simulink model "nonlinearfinal"  (R2021b)
settings: Solver=VariableStepAuto  StartTime=0.0  StopTime=10.0  RelTol=1e-3
libraries: slpidlib x2
settings Model: Creator=Arian  LastModifiedBy=Arian

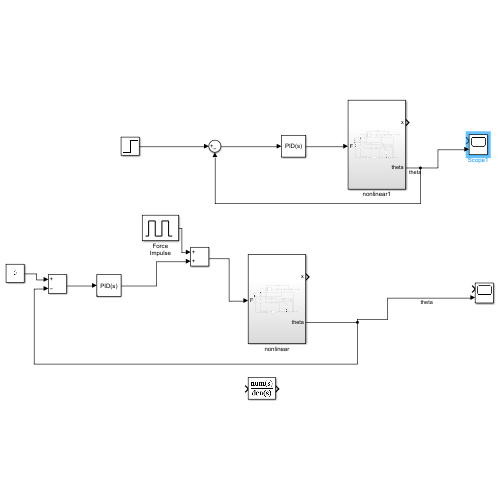
[thumbnail: Simulink's stored preview of the top-level diagram]
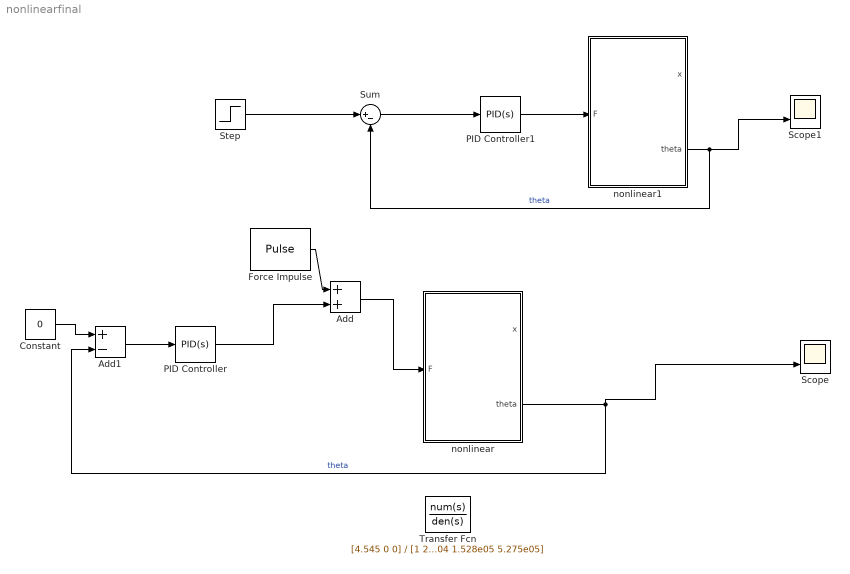
== system nonlinearfinal ==
  Add : Sum
  Add1 : Sum  Inputs=+-
  Constant : Constant  Value=0
  Force Impulse : DiscretePulseGenerator  PulseType=Time based  Amplitude=1000  Period=10  PulseWidth=0.01
  PID Controller : slpidlib/PID Controller  Controller=PID  Form=Parallel  TimeDomain=Continuous-time  UseExternalTs=off  SampleTime=-1  IntegratorMethod=Forward Euler  FilterMethod=Forward Euler  ControllerParametersSource=internal  P=100  I=100  D=20  UseFilter=on  N=1000  TunerSelectOption=Transfer Function Based (PID Tuner App)  InitialConditionSource=internal  InitialConditionForIntegrator=0  InitialConditionForFilter=0  DifferentiatorICPrevScaledInput=0  ExternalReset=none  TrackingMode=off  Kt=1  LimitOutput=off  SatLimitsSource=internal  UpperSaturationLimit=inf  LowerSaturationLimit=-inf  LinearizeAsGain=on  AntiWindupMode=none  Kb=1  POutMin=[]  POutMax=[]  IOutMin=[]  IOutMax=[]  DOutMin=[]  DOutMax=[]  NOutMin=[]  NOutMax=[]  SumOutMin=[]  SumOutMax=[]  SaturationOutMin=[]  SaturationOutMax=[]  PParamMin=[]  PParamMax=[]  IParamMin=[]  IParamMax=[]  DParamMin=[]  DParamMax=[]  NParamMin=[]  NParamMax=[]  KbParamMin=[]  KbParamMax=[]  KtParamMin=[]  KtParamMax=[]  KbOutMin=[]  KbOutMax=[]  KtOutMin=[]  KtOutMax=[]  IntegratorOutMin=[]  IntegratorOutMax=[]  FilterOutMin=[]  FilterOutMax=[]  SumI1OutMin=[]  SumI1OutMax=[]  SumI2OutMin=[]  SumI2OutMax=[]  SumI3OutMin=[]  SumI3OutMax=[]  SumI4OutMin=[]  SumI4OutMax=[]  SumDOutMin=[]  SumDOutMax=[]  DifferentiatorOutMin=[]  DifferentiatorOutMax=[]  FilterDiffOutCoefMin=[]  FilterDiffOutCoefMax=[]  ReciprocalOutMin=[]  ReciprocalOutMax=[]  SumDenOutMin=[]  SumDenOutMax=[]  SumNumOutMin=[]  SumNumOutMax=[]  DivideOutMin=[]  DivideOutMax=[]  UdiffTsProdOutMin=[]  UdiffTsProdOutMax=[]  NTsProdOutMin=[]  NTsProdOutMax=[]  UintegralTsProdOutMin=[]  UintegralTsProdOutMax=[]  UngainTsProdOutMin=[]  UngainTsProdOutMax=[]  IntegratorContinuousStateAttributes=''  IntegratorStateMustResolveToSignalObject=off  IntegratorRTWStateStorageClass=Auto  FilterContinuousStateAttributes=''  FilterStateMustResolveToSignalObject=off  FilterRTWStateStorageClass=Auto  ParallelPVariant=InternalParameters  IdealPVariant=Disabled  IVariant=InternalParameters  DVariant=InternalParameters  IntegratorVariant=Continuous  SatVariant=Disabled  AWVariant=Passthrough  PCopyVariant=Disabled  TRVariant=Disabled  FdbkBlocksVariant=Forward  IdealPFdbkVariant=Disabled  SatFdbkVariant=Disabled  DerivativeFilterVariant=ContFilter  NVariant=InternalParameters  NCopyVariant=Disabled  FilterICVariant=InternalICsFilter  IntegratorICVariant=InternalICs  ExternalResetVariant=Disabled  TRSumVariant=Passthrough  SumFdbkVariant=Disabled  SumVariant=Sum_PID  TsampFilterVariant=InternalTs  TsampNgainVariant=Passthrough  TsampIntegralVariant=Passthrough  ExternalSaturationOutDataTypeStr=Inherit: Same as second input
  PID Controller1 : slpidlib/PID Controller  Controller=PID  Form=Parallel  TimeDomain=Continuous-time  UseExternalTs=off  SampleTime=-1  IntegratorMethod=Forward Euler  FilterMethod=Forward Euler  ControllerParametersSource=internal  P=100  I=100  D=20  UseFilter=on  N=100  TunerSelectOption=Transfer Function Based (PID Tuner App)  InitialConditionSource=internal  InitialConditionForIntegrator=0  InitialConditionForFilter=0  DifferentiatorICPrevScaledInput=0  ExternalReset=none  TrackingMode=off  Kt=1  LimitOutput=off  SatLimitsSource=internal  UpperSaturationLimit=inf  LowerSaturationLimit=-inf  LinearizeAsGain=on  AntiWindupMode=none  Kb=1  POutMin=[]  POutMax=[]  IOutMin=[]  IOutMax=[]  DOutMin=[]  DOutMax=[]  NOutMin=[]  NOutMax=[]  SumOutMin=[]  SumOutMax=[]  SaturationOutMin=[]  SaturationOutMax=[]  PParamMin=[]  PParamMax=[]  IParamMin=[]  IParamMax=[]  DParamMin=[]  DParamMax=[]  NParamMin=[]  NParamMax=[]  KbParamMin=[]  KbParamMax=[]  KtParamMin=[]  KtParamMax=[]  KbOutMin=[]  KbOutMax=[]  KtOutMin=[]  KtOutMax=[]  IntegratorOutMin=[]  IntegratorOutMax=[]  FilterOutMin=[]  FilterOutMax=[]  SumI1OutMin=[]  SumI1OutMax=[]  SumI2OutMin=[]  SumI2OutMax=[]  SumI3OutMin=[]  SumI3OutMax=[]  SumI4OutMin=[]  SumI4OutMax=[]  SumDOutMin=[]  SumDOutMax=[]  DifferentiatorOutMin=[]  DifferentiatorOutMax=[]  FilterDiffOutCoefMin=[]  FilterDiffOutCoefMax=[]  ReciprocalOutMin=[]  ReciprocalOutMax=[]  SumDenOutMin=[]  SumDenOutMax=[]  SumNumOutMin=[]  SumNumOutMax=[]  DivideOutMin=[]  DivideOutMax=[]  UdiffTsProdOutMin=[]  UdiffTsProdOutMax=[]  NTsProdOutMin=[]  NTsProdOutMax=[]  UintegralTsProdOutMin=[]  UintegralTsProdOutMax=[]  UngainTsProdOutMin=[]  UngainTsProdOutMax=[]  IntegratorContinuousStateAttributes=''  IntegratorStateMustResolveToSignalObject=off  IntegratorRTWStateStorageClass=Auto  FilterContinuousStateAttributes=''  FilterStateMustResolveToSignalObject=off  FilterRTWStateStorageClass=Auto  ParallelPVariant=InternalParameters  IdealPVariant=Disabled  IVariant=InternalParameters  DVariant=InternalParameters  IntegratorVariant=Continuous  SatVariant=Disabled  AWVariant=Passthrough  PCopyVariant=Disabled  TRVariant=Disabled  FdbkBlocksVariant=Forward  IdealPFdbkVariant=Disabled  SatFdbkVariant=Disabled  DerivativeFilterVariant=ContFilter  NVariant=InternalParameters  NCopyVariant=Disabled  FilterICVariant=InternalICsFilter  IntegratorICVariant=InternalICs  ExternalResetVariant=Disabled  TRSumVariant=Passthrough  SumFdbkVariant=Disabled  SumVariant=Sum_PID  TsampFilterVariant=InternalTs  TsampNgainVariant=Passthrough  TsampIntegralVariant=Passthrough  ExternalSaturationOutDataTypeStr=Inherit: Same as second input
  Scope : Scope  NumInputPorts=2
  Scope1 : Scope  NumInputPorts=2
  Step : Step  SampleTime=0
  Sum : Sum  Inputs=|+-
  Transfer Fcn : TransferFcn  Numerator=[4.545 0 0]  Denominator=[1 250 1.68e04 1.528e05 5.275e05]
  nonlinear : Subsystem
  nonlinear1 : Subsystem
  wires:
  nonlinear1/2(theta) -> Scope1/2, Sum/2  "theta"
  PID Controller1/1 -> nonlinear1/1(F)
  Sum/1 -> PID Controller1/1
  Step/1 -> Sum/1
  Add1/1 -> PID Controller/1
  Constant/1 -> Add1/1
  Add/1 -> nonlinear/1(F)
  PID Controller/1 -> Add/2
  Force Impulse/1 -> Add/1
  nonlinear/2(theta) -> Scope/2, Add1/2  "theta"

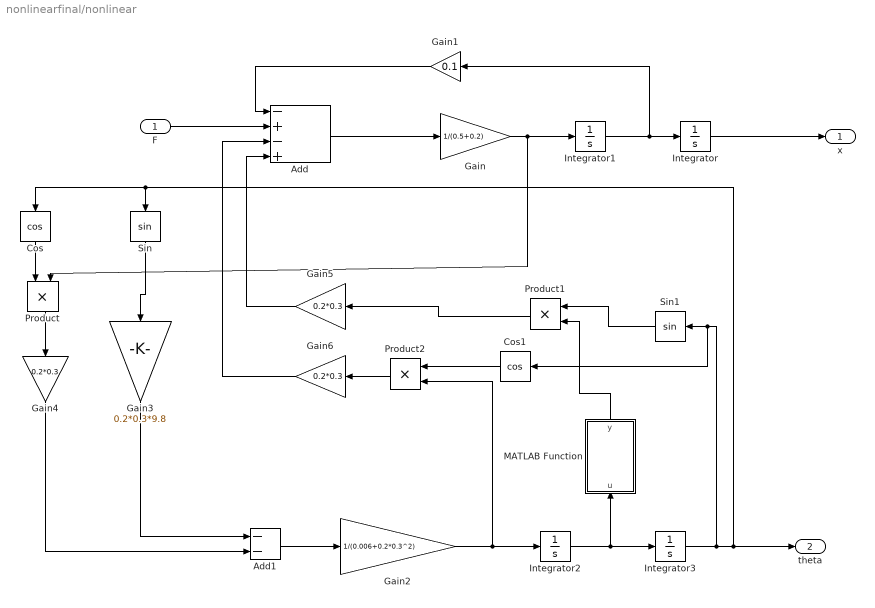
== system nonlinearfinal/nonlinear ==
  F : Inport
  Add : Sum  Inputs=-+-+
  Add1 : Sum  Inputs=--
  Cos : Trigonometry  Operator=cos
  Cos1 : Trigonometry  Operator=cos
  Gain : Gain  Gain=1/(0.5+0.2)
  Gain1 : Gain  Gain=0.1
  Gain2 : Gain  Gain=1/(0.006+0.2*0.3^2)
  Gain3 : Gain  Gain=0.2*0.3*9.8
  Gain4 : Gain  Gain=0.2*0.3
  Gain5 : Gain  Gain=0.2*0.3
  Gain6 : Gain  Gain=0.2*0.3
  Integrator{,1..3} (4 alike) : Integrator
  MATLAB Function : MATLAB Function  TreatAsAtomicUnit=on
  Product : Product
  Product1 : Product
  Product2 : Product
  Sin : Trigonometry
  Sin1 : Trigonometry
  x : Outport
  theta : Outport  Port=2
  wires:
  Integrator3/1 -> Cos1/1, Sin1/1, theta/1, Cos/1, Sin/1
  MATLAB Function/1(y) -> Product1/2
  Gain1/1 -> Add/1
  Add/1 -> Gain/1
  Integrator2/1 -> Integrator3/1, MATLAB Function/1(u)
  Product2/1 -> Gain6/1
  Gain/1 -> Product/2, Integrator1/1
  Cos/1 -> Product/1
  Gain2/1 -> Product2/2, Integrator2/1
  Integrator/1 -> x/1
  Integrator1/1 -> Gain1/1, Integrator/1
  Cos1/1 -> Product2/1
  Gain5/1 -> Add/4
  Product1/1 -> Gain5/1
  F/1 -> Add/2
  Sin/1 -> Gain3/1
  Sin1/1 -> Product1/1
  Gain4/1 -> Add1/2
  Gain3/1 -> Add1/1
  Product/1 -> Gain4/1
  Gain6/1 -> Add/3
  Add1/1 -> Gain2/1

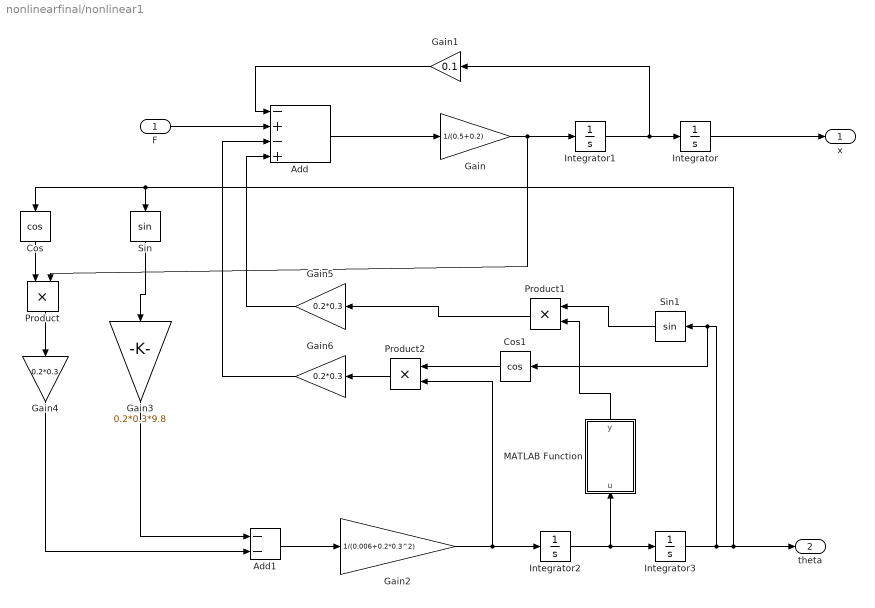
== system nonlinearfinal/nonlinear1 ==
  F : Inport
  Add : Sum  Inputs=-+-+
  Add1 : Sum  Inputs=--
  Cos : Trigonometry  Operator=cos
  Cos1 : Trigonometry  Operator=cos
  Gain : Gain  Gain=1/(0.5+0.2)
  Gain1 : Gain  Gain=0.1
  Gain2 : Gain  Gain=1/(0.006+0.2*0.3^2)
  Gain3 : Gain  Gain=0.2*0.3*9.8
  Gain4 : Gain  Gain=0.2*0.3
  Gain5 : Gain  Gain=0.2*0.3
  Gain6 : Gain  Gain=0.2*0.3
  Integrator{,1..3} (4 alike) : Integrator
  MATLAB Function : MATLAB Function  TreatAsAtomicUnit=on
  Product : Product
  Product1 : Product
  Product2 : Product
  Sin : Trigonometry
  Sin1 : Trigonometry
  x : Outport
  theta : Outport  Port=2
  wires:
  Integrator3/1 -> Cos1/1, Sin1/1, theta/1, Cos/1, Sin/1
  MATLAB Function/1(y) -> Product1/2
  Gain1/1 -> Add/1
  Add/1 -> Gain/1
  Integrator2/1 -> Integrator3/1, MATLAB Function/1(u)
  Product2/1 -> Gain6/1
  Gain/1 -> Product/2, Integrator1/1
  Cos/1 -> Product/1
  Gain2/1 -> Product2/2, Integrator2/1
  Integrator/1 -> x/1
  Integrator1/1 -> Gain1/1, Integrator/1
  Cos1/1 -> Product2/1
  Gain5/1 -> Add/4
  Product1/1 -> Gain5/1
  F/1 -> Add/2
  Sin/1 -> Gain3/1
  Sin1/1 -> Product1/1
  Gain4/1 -> Add1/2
  Gain3/1 -> Add1/1
  Product/1 -> Gain4/1
  Gain6/1 -> Add/3
  Add1/1 -> Gain2/1

== matlab function nonlinearfinal/nonlinear/MATLAB Function ==
  data: u input; y output
function y = fcn(u)

y = u*u;

== matlab function nonlinearfinal/nonlinear1/MATLAB Function ==
  data: u input; y output
function y = fcn(u)

y = u*u;
